simulink model "Interleaving_Buck_Boost"  (R2022a)
settings: Solver=VariableStepAuto  StartTime=0.0  StopTime=1  RelTol=1e-3
libraries: spsSeriesRLCBranchLib x6, spsCurrentMeasurementLib x2, spsDiodeLib x2, spsMosfetLib x2, spsVoltageMeasurementLib x2, spsDCVoltageSourceLib x1, spsMultimeterLib x1, spspowerguiLib x1
settings Model: Creator=Bobby  LastModifiedBy=Bobby

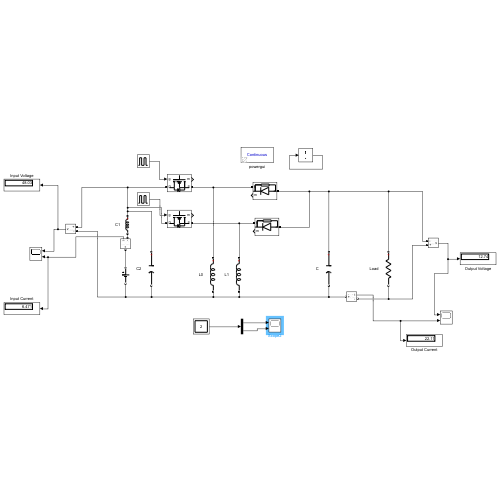
[thumbnail: Simulink's stored preview of the top-level diagram]
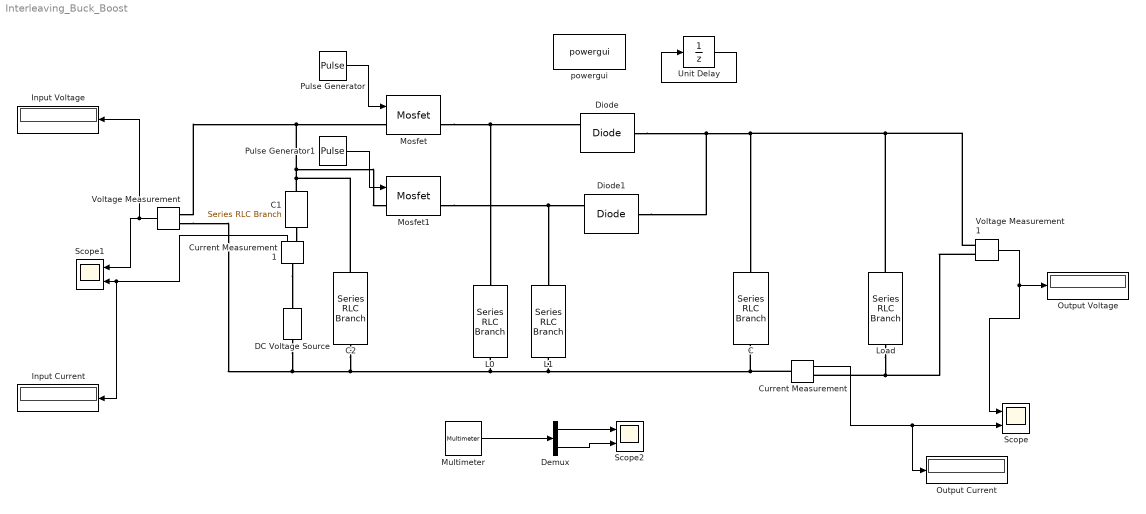
== system Interleaving_Buck_Boost ==
  C : spsSeriesRLCBranchLib/Series RLC Branch  LConnTagsString=__new0  RConnTagsString=__new0  BranchType=C  Resistance=1  Inductance=1e-3  SetiL0=off  InitialCurrent=0  Capacitance=1.667e-3  Setx0=off  InitialVoltage=0  Measurements=None
  C1 : spsSeriesRLCBranchLib/Series RLC Branch  LConnTagsString=__new0  RConnTagsString=__new0  BranchType=L  Resistance=0.001  Inductance=220e-6  SetiL0=off  InitialCurrent=0  Capacitance=200e-6  Setx0=off  InitialVoltage=0  Measurements=None
  C2 : spsSeriesRLCBranchLib/Series RLC Branch  LConnTagsString=__new0  RConnTagsString=__new0  BranchType=C  Resistance=0.001  Inductance=1e-3  SetiL0=off  InitialCurrent=0  Capacitance=470e-6  Setx0=off  InitialVoltage=0  Measurements=None
  Current Measurement : spsCurrentMeasurementLib/Current Measurement  PhasorSimulation=off  OutputType=Complex  PSBequivalent=0
  Current Measurement1 : spsCurrentMeasurementLib/Current Measurement  PhasorSimulation=off  OutputType=Complex  PSBequivalent=0
  DC Voltage Source : spsDCVoltageSourceLib/DC Voltage Source  Amplitude=48  Measurements=None
  Demux : Demux  Outputs=2
  Diode : spsDiodeLib/Diode  Ron=0.001  Lon=0  Vf=0.8  IC=0  UseSnubber=0  Rs=500  Cs=250e-9  Measurements=on
  Diode1 : spsDiodeLib/Diode  Ron=0.001  Lon=0  Vf=0.8  IC=0  UseSnubber=0  Rs=500  Cs=250e-9  Measurements=on
  Input Current : Display
  Input Voltage : Display
  L0 : spsSeriesRLCBranchLib/Series RLC Branch  LConnTagsString=__new0  RConnTagsString=__new0  BranchType=L  Resistance=1  Inductance=64e-6  SetiL0=off  InitialCurrent=0  Capacitance=1e-6  Setx0=off  InitialVoltage=0  Measurements=Branch current
  L1 : spsSeriesRLCBranchLib/Series RLC Branch  LConnTagsString=__new0  RConnTagsString=__new0  BranchType=L  Resistance=1  Inductance=64e-6  SetiL0=off  InitialCurrent=0  Capacitance=1e-6  Setx0=off  InitialVoltage=0  Measurements=Branch current
  Load : spsSeriesRLCBranchLib/Series RLC Branch  LConnTagsString=__new0  RConnTagsString=__new0  BranchType=R  Resistance=0.576  Inductance=1e-3  SetiL0=off  InitialCurrent=0  Capacitance=1e-6  Setx0=off  InitialVoltage=0  Measurements=None
  Mosfet : spsMosfetLib/Mosfet  Ron=0.1  Lon=0  Rd=0.01  Vfd=0  IC=0  Rs=1e5  Cs=inf  Measurements=on
  Mosfet1 : spsMosfetLib/Mosfet  Ron=0.1  Lon=0  Rd=0.01  Vfd=0  IC=0  Rs=1e5  Cs=inf  Measurements=on
  Multimeter : spsMultimeterLib/Multimeter  L=2  sel=[1 2]  yselected={}  Gain=[1 1]  OutputType=Complex  PlotAtSimulationStop=off  PhasorSimulation=off
  Output Current : Display
  Output Voltage : Display
  Pulse Generator : DiscretePulseGenerator  PulseType=Time based  Period=2e-5  PulseWidth=22.5
  Pulse Generator1 : DiscretePulseGenerator  PulseType=Time based  Period=20e-6  PulseWidth=22.5  PhaseDelay=10e-6
  Scope : Scope  NumInputPorts=2
  Scope1 : Scope  NumInputPorts=2
  Scope2 : Scope  NumInputPorts=2
  Unit Delay : UnitDelay  SampleTime=-1  HasFrameUpgradeWarning=on
  Voltage Measurement : spsVoltageMeasurementLib/Voltage Measurement  PhasorSimulation=off  OutputType=Complex  PSBequivalent=0
  Voltage Measurement1 : spsVoltageMeasurementLib/Voltage Measurement  PhasorSimulation=off  OutputType=Complex  PSBequivalent=0
  powergui : spspowerguiLib/powergui  Priority=1  SimulationMode=Continuous  SampleTime=50e-6  frequency=60  Iterations=50  frequencyindice=0  Pbase=100e6  ErrMax=1e-4  UnitsV=kV  UnitsW=MW  buscounter=0  FunctionMessages=off  echomessages=off  EnableUseOfTLC=off  CurrentSourceSwitches=off  DisableSnubberDevices=off  DisableRonSwitches=off  DisableVfSwitches=off  DisplayEquations=off  AutomaticDiscreteSolvers=off  SolverType=Tustin/Backward Euler (TBE)  Interpol=off  ExternalGateDelay=off  methode=off  Ts=100  x0status=blocks  SPID=on  SwTol=0  HookPort=off  NonlinearTolerance=1e-4  nMaxIteration=100  ContinueOnMaxIteration=off  RestoreLinks=warning  ResistiveCurrentMeasurement=off  Frange=[0:2:500]  Ylog=off  Xlog=on  ShowGrid=off  save=off  variable=ZData  structure=0  ZoomFFT=off  StartTime=0.0  cycles=1  DisplayStyle=1  fundamental=60  FreqAxis=off  MaxFrequency=1000  frequencyindicesteady=1  RmsSteady=1  display=off
  wires:
  Pulse Generator/1 -> Mosfet/1
  Pulse Generator1/1 -> Mosfet1/1
  Voltage Measurement/1 -> Input Voltage/1, Scope1/1
  Unit Delay/1 -> Unit Delay/1
  Current Measurement/1 -> Output Current/1, Scope/2
  Voltage Measurement1/1 -> Output Voltage/1, Scope/1
  Multimeter/1 -> Demux/1
  Demux/1 -> Scope2/1
  Demux/2 -> Scope2/2
  Current Measurement1/1 -> Input Current/1, Scope1/2
  connections:
  Mosfet/RConn1 -- L0/LConn1 -- Diode/RConn1
  Mosfet1/RConn1 -- L1/LConn1 -- Diode1/RConn1
  Diode/LConn1 -- Diode1/LConn1 -- Load/LConn1 -- Voltage Measurement1/LConn2 -- C/LConn1
  DC Voltage Source/LConn1 -- Voltage Measurement/LConn2 -- C2/RConn1 -- Current Measurement/LConn1 -- C/RConn1 -- L1/RConn1 -- L0/RConn1
  Load/RConn1 -- Voltage Measurement1/LConn1 -- Current Measurement/RConn1
  Voltage Measurement/LConn1 -- C2/LConn1 -- C1/LConn1 -- Mosfet1/LConn1 -- Mosfet/LConn1
  Current Measurement1/LConn1 -- DC Voltage Source/RConn1
  C1/RConn1 -- Current Measurement1/RConn1
